simulink model "Lab3_compensator"  (R2025b)
settings: Solver=ode45  StartTime=0.0  StopTime=150  MaxStep=0.005  RelTol=1e-3
values from neighbouring files (symbols this model uses):
  A = 14.1208    [lab_3_simulation.m]    (also in lab_simulation.m)
  Ascale = 1    [lab_3_simulation.m]    (also in lab_simulation.m)
  delta = 0.0014    [lab_3_simulation.m]    (also in lab_simulation.m)
  distSize = 0    [lab_3_simulation.m]    (also in lab_simulation.m)
  distTime = 40    [lab_3_simulation.m]    (also in lab_simulation.m)
  hover = 2.5    [lab_3_simulation.m]    (also in lab_simulation.m)
  k_theta = 1.0    (= 1)    [lab_simulation.m]
  Kc = 0.711    [lab_3_simulation.m]    (also in lab_simulation.m = 0.713)
  ks = 0.6599    [lab_3_simulation.m]    (also in lab_simulation.m)
  p = 1.000    (= 1)    [lab_3_simulation.m]    (also in lab_simulation.m)
  rFinal = 0    [lab_3_simulation.m]    (also in lab_simulation.m)
  sineAmp = 1    [lab_3_simulation.m]    (also in lab_simulation.m)
  tau = 12.9898    [lab_3_simulation.m]    (also in lab_simulation.m)
  tauScale = 1    [lab_3_simulation.m]    (also in lab_simulation.m)
  z = b    (= 0.0769834793453)    [lab_3_simulation.m]    (also in lab_simulation.m = 0.0770617881417)
settings Model: Creator=MTMTAD006  LastModifiedBy=MTMTAD006

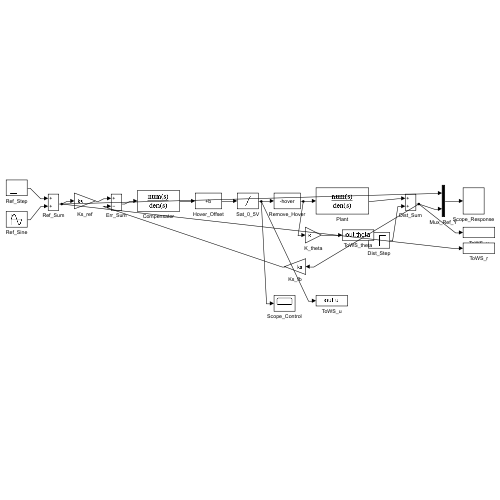
[thumbnail: Simulink's stored preview of the top-level diagram]
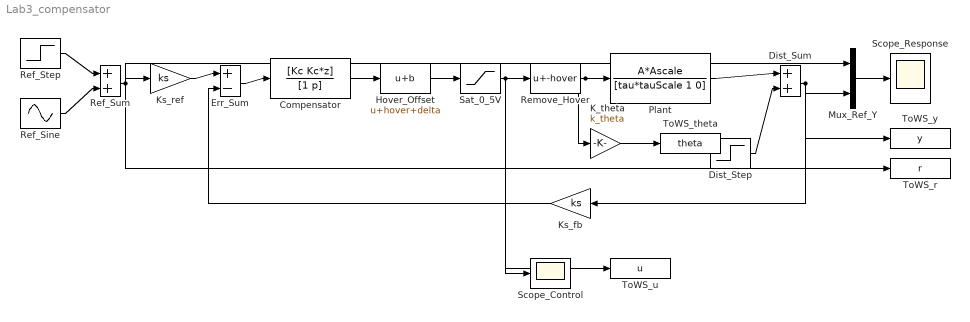
== system Lab3_compensator ==
  Compensator : TransferFcn  Numerator=[Kc Kc*z]  Denominator=[1 p]
  Dist_Step : Step  Time=distTime  After=distSize  SampleTime=0
  Dist_Sum : Sum
  Err_Sum : Sum  Inputs=+-
  Hover_Offset : Bias  Bias=hover+delta  SaturateOnIntegerOverflow=off
  K_theta : Gain  Gain=k_theta
  Ks_fb : Gain  Gain=ks
  Ks_ref : Gain  Gain=ks
  Mux_Ref_Y : Mux  Inputs=2
  Plant : TransferFcn  Numerator=A*Ascale  Denominator=[tau*tauScale 1 0]
  Ref_Sine : Sin  Amplitude=sineAmp  Frequency=0.1  SampleTime=0
  Ref_Step : Step  Time=0  After=rFinal  SampleTime=0
  Ref_Sum : Sum
  Remove_Hover : Bias  Bias=-hover  SaturateOnIntegerOverflow=off
  Sat_0_5V : Saturate  UpperLimit=5  LowerLimit=0
  Scope_Control : Scope
  Scope_Response : Scope
  ToWS_r : ToWorkspace  VariableName=r  SampleTime=-1
  ToWS_theta : ToWorkspace  VariableName=theta  SampleTime=-1
  ToWS_u : ToWorkspace  VariableName=u  SampleTime=-1
  ToWS_y : ToWorkspace  VariableName=y  SampleTime=-1
  wires:
  Ref_Step/1 -> Ref_Sum/1
  Ref_Sine/1 -> Ref_Sum/2
  Ref_Sum/1 -> Ks_ref/1, Mux_Ref_Y/1, ToWS_r/1
  Ks_ref/1 -> Err_Sum/1
  Ks_fb/1 -> Err_Sum/2
  Err_Sum/1 -> Compensator/1
  Compensator/1 -> Hover_Offset/1
  Hover_Offset/1 -> Sat_0_5V/1
  Sat_0_5V/1 -> Remove_Hover/1, Scope_Control/1, ToWS_u/1
  Remove_Hover/1 -> Plant/1, K_theta/1
  K_theta/1 -> ToWS_theta/1
  Plant/1 -> Dist_Sum/1
  Dist_Step/1 -> Dist_Sum/2
  Dist_Sum/1 -> Ks_fb/1, Mux_Ref_Y/2, ToWS_y/1
  Mux_Ref_Y/1 -> Scope_Response/1
